simulink model "ElectricVehicleThermalManagementWithHeatPump_2026a_version"  (R2026a)
settings: Solver=VariableStepAuto  StopTime=3600  AbsTol=1e-3
PreLoadFcn:
  | init_nmpc
InitFcn:
  | init_nmpc
model workspace: external: MATLAB File ElectricVehicleThermalManagementWithHeatPumpParameters.m (data not in the file)
values from neighbouring files (symbols this model uses):
  battery_C1_LUT = [1913.6 12447 30609 ... (first row only)    [ElectricVehicleThermalManagementWithHeatPumpParameters.m]
  battery_capacity_LUT = [280.081 276.25 276.392]    [ElectricVehicleThermalManagementWithHeatPumpParameters.m]
  battery_cell_cp = 795    [ElectricVehicleThermalManagementWithHeatPumpParameters.m]
  battery_cell_mass = 2.5    [ElectricVehicleThermalManagementWithHeatPumpParameters.m]
  battery_Em_LUT = [3.4966 3.5057 3.5148 ... (first row only)    [ElectricVehicleThermalManagementWithHeatPumpParameters.m]
  battery_N_cells = 20    [ElectricVehicleThermalManagementWithHeatPumpParameters.m]
  battery_Qe_init = 0    [ElectricVehicleThermalManagementWithHeatPumpParameters.m]
  battery_R0_LUT = [0.0117 0.0085 0.009 ... (first row only)    [ElectricVehicleThermalManagementWithHeatPumpParameters.m]
  battery_R1_LUT = [0.0109 0.0029 0.0013 ... (first row only)    [ElectricVehicleThermalManagementWithHeatPumpParameters.m]
  battery_SOC_LUT = [0; 0.1; 0.25; 0.5; 0.75; 0.9; 1]    [ElectricVehicleThermalManagementWithHeatPumpParameters.m]
  battery_T_init = -5    [ElectricVehicleThermalManagementWithHeatPumpParameters.m]
  battery_temperature_LUT = [5 20 40]    [ElectricVehicleThermalManagementWithHeatPumpParameters.m]
  cabin_duct_area = 0.04    [ElectricVehicleThermalManagementWithHeatPumpParameters.m]
  cabin_T_init = -5    [ElectricVehicleThermalManagementWithHeatPumpParameters.m]
  chiller_area_primary = 0.43982297150257105    (= 0.439822971503)    [ElectricVehicleThermalManagementWithHeatPumpParameters.m]
  chiller_N_baffles = 3    [ElectricVehicleThermalManagementWithHeatPumpParameters.m]
  chiller_N_tubes = 100    [ElectricVehicleThermalManagementWithHeatPumpParameters.m]
  chiller_tube_D = 0.0035    [ElectricVehicleThermalManagementWithHeatPumpParameters.m]
  chiller_tube_L = 0.4    [ElectricVehicleThermalManagementWithHeatPumpParameters.m]
  chiller_wall_conductivity = 240    [ElectricVehicleThermalManagementWithHeatPumpParameters.m]
  chiller_wall_thickness = 0.0001    [ElectricVehicleThermalManagementWithHeatPumpParameters.m]
  cond_evap_air_area_flow = 0.3906    [ElectricVehicleThermalManagementWithHeatPumpParameters.m]
  cond_evap_air_area_primary = 1.4834999999999998    (= 1.4835)    [ElectricVehicleThermalManagementWithHeatPumpParameters.m]
  cond_evap_W = 0.015    [ElectricVehicleThermalManagementWithHeatPumpParameters.m]
  cond_evap_wall_conductivity = 240    [ElectricVehicleThermalManagementWithHeatPumpParameters.m]
  cond_evap_wall_thickness = 0.0001    [ElectricVehicleThermalManagementWithHeatPumpParameters.m]
  coolant_channel_D = 0.0092    [ElectricVehicleThermalManagementWithHeatPumpParameters.m]
  coolant_pipe_D = 0.019    [ElectricVehicleThermalManagementWithHeatPumpParameters.m]
  coolant_T_init = -5    [ElectricVehicleThermalManagementWithHeatPumpParameters.m]
  coolant_tank_area = 0.0121    [ElectricVehicleThermalManagementWithHeatPumpParameters.m]
  coolant_tank_volume = 1.25    [ElectricVehicleThermalManagementWithHeatPumpParameters.m]
  coolant_valve_D_ratio_max = 0.95    [ElectricVehicleThermalManagementWithHeatPumpParameters.m]
  coolant_valve_D_ratio_min = 0.001    [ElectricVehicleThermalManagementWithHeatPumpParameters.m]
  coolant_valve_displacement = 0.0063    [ElectricVehicleThermalManagementWithHeatPumpParameters.m]
  coolant_valve_S_max = 0.0053    [ElectricVehicleThermalManagementWithHeatPumpParameters.m]
  evaporator_air_area_flow = 0.12    [ElectricVehicleThermalManagementWithHeatPumpParameters.m]
  evaporator_air_area_primary = 0.4323    [ElectricVehicleThermalManagementWithHeatPumpParameters.m]
  evaporator_W = 0.015    [ElectricVehicleThermalManagementWithHeatPumpParameters.m]
  evaporator_wall_conductivity = 240    [ElectricVehicleThermalManagementWithHeatPumpParameters.m]
  evaporator_wall_thickness = 0.0001    [ElectricVehicleThermalManagementWithHeatPumpParameters.m]
  expansion_valve_D_ratio_max = 0.9    [ElectricVehicleThermalManagementWithHeatPumpParameters.m]
  hex_area_primary = 0.070371675440411369    (= 0.0703716754404)    [ElectricVehicleThermalManagementWithHeatPumpParameters.m]
  hex_N_tubes = 64    [ElectricVehicleThermalManagementWithHeatPumpParameters.m]
  hex_tube_D = 0.0035    [ElectricVehicleThermalManagementWithHeatPumpParameters.m]
  hex_wall_conductivity = 240    [ElectricVehicleThermalManagementWithHeatPumpParameters.m]
  hex_wall_thickness = 0.0001    [ElectricVehicleThermalManagementWithHeatPumpParameters.m]
  inner_cond_air_area_flow = 0.1953    [ElectricVehicleThermalManagementWithHeatPumpParameters.m]
  inner_cond_air_area_primary = 0.99520000000000008    (= 0.9952)    [ElectricVehicleThermalManagementWithHeatPumpParameters.m]
  inner_cond_W = 0.02    [ElectricVehicleThermalManagementWithHeatPumpParameters.m]
  inner_cond_wall_conductivity = 240    [ElectricVehicleThermalManagementWithHeatPumpParameters.m]
  inner_cond_wall_thickness = 0.0001    [ElectricVehicleThermalManagementWithHeatPumpParameters.m]
  pump_speed_max = 1000    [ElectricVehicleThermalManagementWithHeatPumpParameters.m]
  radiator_air_area_flow = 0.097499999999999989    (= 0.0975)    [ElectricVehicleThermalManagementWithHeatPumpParameters.m]
  radiator_air_area_primary = 0.43687499999999996    (= 0.436875)    [ElectricVehicleThermalManagementWithHeatPumpParameters.m]
  radiator_W = 0.015    [ElectricVehicleThermalManagementWithHeatPumpParameters.m]
  radiator_wall_conductivity = 240    [ElectricVehicleThermalManagementWithHeatPumpParameters.m]
  radiator_wall_thickness = 0.0001    [ElectricVehicleThermalManagementWithHeatPumpParameters.m]
  refrigerant_p_init = 0.25    [ElectricVehicleThermalManagementWithHeatPumpParameters.m]
  refrigerant_pipe_D = 0.01    [ElectricVehicleThermalManagementWithHeatPumpParameters.m]
  refrigerant_valve_D_ratio_max = 0.95    [ElectricVehicleThermalManagementWithHeatPumpParameters.m]
  refrigerant_valve_displacement = 0.005    [ElectricVehicleThermalManagementWithHeatPumpParameters.m]
libraries: fl_lib x227, nesl_utility x162, SimscapeFluids_lib x30, LiBatteryElements_lib x16, slpidlib x3, SignalEditorBlockLib x1
(part 12 of 13)

== system ElectricVehicleThermalManagementWithHeatPump_2026a_version/Battery/Pack 2/Thermal Model ==
  Battery Thermal Mass : fl_lib/Thermal/Thermal Elements/Thermal Mass  mass_type=foundation.enum.constant_variable.constant  mass=cell_mass*Ncells kg  sp_heat=cell_Cp_heat J/kg/K  mass_min=1e-6 kg  num_ports=foundation.enum.numPorts2.one  m_specify=off  m_priority=High  m=1 kg  m_nominal_specify=off  m_nominal_value=1  m_nominal_unit=kg  T_specify=on  T_priority=High  T=T_init K  T_nominal_specify=off  T_nominal_value=1  T_nominal_unit=K  Q_specify=off  Q_priority=None  Q=0 W  Q_nominal_specify=off  Q_nominal_value=1  Q_nominal_unit=W
  Controlled Heat Flow Rate Source : fl_lib/Thermal/Thermal Sources/Controlled Heat Flow Rate Source
  Temperature Sensor : fl_lib/Thermal/Thermal Sensors/Temperature Sensor  temperature_measure=foundation.enum.MeasurementReference.difference
  Thermal Reference : fl_lib/Thermal/Thermal Elements/Thermal Reference
  Thermal Reference2 : fl_lib/Thermal/Thermal Elements/Thermal Reference
  H : PMIOPort  Side=Left
  Pxn : PMIOPort  Port=2  Side=Left
  T : PMIOPort  Port=3  Side=Right
  connections:
  H/RConn1 -- Controlled Heat Flow Rate Source/LConn1 -- Battery Thermal Mass/LConn1 -- Temperature Sensor/LConn1
  Pxn/RConn1 -- Controlled Heat Flow Rate Source/RConn1
  Controlled Heat Flow Rate Source/RConn2 -- Thermal Reference2/LConn1
  Thermal Reference/LConn1 -- Temperature Sensor/RConn1
  T/RConn1 -- Temperature Sensor/RConn2

== system ElectricVehicleThermalManagementWithHeatPump_2026a_version/Battery/Pack 3/Lithium Cell 1RC ==
  note: Power
      | Losses
  C1 : LiBatteryElements_lib/C_table  C_Table=C1_LUT F  SOC_Table=SOC_LUT  Temp_Table=Temperature_LUT K  v0=0 V
  Em_table : LiBatteryElements_lib/Em_table  C_Table=Capacity_LUT hr*A  Em_Table=Em_LUT V  SOC_Table=SOC_LUT  Temp_Table=Temperature_LUT K  Qinit=Qe_init hr*A
  Power Sum : fl_lib/Physical Signals/Functions/PS Add
  R0 : LiBatteryElements_lib/R_table  R_Table=R0_LUT Ohm  SOC_Table=SOC_LUT  Temp_Table=Temperature_LUT K
  R1 : LiBatteryElements_lib/R_table  R_Table=R1_LUT Ohm  SOC_Table=SOC_LUT  Temp_Table=Temperature_LUT K
  P : PMIOPort  Side=Left
  + : PMIOPort  Port=2  Side=Left
  T : PMIOPort  Port=3  Side=Right
  - : PMIOPort  Port=4  Side=Right
  connections:
  R0/LConn3 -- R1/LConn3 -- Em_table/LConn3 -- C1/LConn3
  Em_table/RConn1 -- -/RConn1
  R0/LConn1 -- R1/RConn1 -- C1/RConn1
  R1/LConn1 -- C1/LConn1 -- Em_table/LConn1
  R1/LConn2 -- C1/LConn2 -- R0/LConn2 -- Em_table/RConn2 -- T/RConn1
  +/RConn1 -- R0/RConn1
  P/RConn1 -- Power Sum/RConn1
  Power Sum/LConn2 -- R0/RConn2
  R1/RConn2 -- Power Sum/LConn1

== system ElectricVehicleThermalManagementWithHeatPump_2026a_version/Battery/Pack 3/Thermal Model ==
  Battery Thermal Mass : fl_lib/Thermal/Thermal Elements/Thermal Mass  mass_type=foundation.enum.constant_variable.constant  mass=cell_mass*Ncells kg  sp_heat=cell_Cp_heat J/kg/K  mass_min=1e-6 kg  num_ports=foundation.enum.numPorts2.one  m_specify=off  m_priority=High  m=1 kg  m_nominal_specify=off  m_nominal_value=1  m_nominal_unit=kg  T_specify=on  T_priority=High  T=T_init K  T_nominal_specify=off  T_nominal_value=1  T_nominal_unit=K  Q_specify=off  Q_priority=None  Q=0 W  Q_nominal_specify=off  Q_nominal_value=1  Q_nominal_unit=W
  Controlled Heat Flow Rate Source : fl_lib/Thermal/Thermal Sources/Controlled Heat Flow Rate Source
  Temperature Sensor : fl_lib/Thermal/Thermal Sensors/Temperature Sensor  temperature_measure=foundation.enum.MeasurementReference.difference
  Thermal Reference : fl_lib/Thermal/Thermal Elements/Thermal Reference
  Thermal Reference2 : fl_lib/Thermal/Thermal Elements/Thermal Reference
  H : PMIOPort  Side=Left
  Pxn : PMIOPort  Port=2  Side=Left
  T : PMIOPort  Port=3  Side=Right
  connections:
  T/RConn1 -- Temperature Sensor/RConn2
  Thermal Reference/LConn1 -- Temperature Sensor/RConn1
  Controlled Heat Flow Rate Source/RConn2 -- Thermal Reference2/LConn1
  Pxn/RConn1 -- Controlled Heat Flow Rate Source/RConn1
  Temperature Sensor/LConn1 -- Battery Thermal Mass/LConn1 -- Controlled Heat Flow Rate Source/LConn1 -- H/RConn1

== system ElectricVehicleThermalManagementWithHeatPump_2026a_version/Battery/Pack 4/Lithium Cell 1RC ==
  note: Power
      | Losses
  C1 : LiBatteryElements_lib/C_table  C_Table=C1_LUT F  SOC_Table=SOC_LUT  Temp_Table=Temperature_LUT K  v0=0 V
  Em_table : LiBatteryElements_lib/Em_table  C_Table=Capacity_LUT hr*A  Em_Table=Em_LUT V  SOC_Table=SOC_LUT  Temp_Table=Temperature_LUT K  Qinit=Qe_init hr*A
  Power Sum : fl_lib/Physical Signals/Functions/PS Add
  R0 : LiBatteryElements_lib/R_table  R_Table=R0_LUT Ohm  SOC_Table=SOC_LUT  Temp_Table=Temperature_LUT K
  R1 : LiBatteryElements_lib/R_table  R_Table=R1_LUT Ohm  SOC_Table=SOC_LUT  Temp_Table=Temperature_LUT K
  P : PMIOPort  Side=Left
  + : PMIOPort  Port=2  Side=Left
  T : PMIOPort  Port=3  Side=Right
  - : PMIOPort  Port=4  Side=Right
  connections:
  R1/RConn2 -- Power Sum/LConn1
  Power Sum/LConn2 -- R0/RConn2
  P/RConn1 -- Power Sum/RConn1
  +/RConn1 -- R0/RConn1
  T/RConn1 -- Em_table/RConn2 -- R0/LConn2 -- C1/LConn2 -- R1/LConn2
  Em_table/LConn1 -- C1/LConn1 -- R1/LConn1
  C1/RConn1 -- R1/RConn1 -- R0/LConn1
  Em_table/RConn1 -- -/RConn1
  C1/LConn3 -- Em_table/LConn3 -- R1/LConn3 -- R0/LConn3

== system ElectricVehicleThermalManagementWithHeatPump_2026a_version/Battery/Pack 4/Thermal Model ==
  Battery Thermal Mass : fl_lib/Thermal/Thermal Elements/Thermal Mass  mass_type=foundation.enum.constant_variable.constant  mass=cell_mass*Ncells kg  sp_heat=cell_Cp_heat J/kg/K  mass_min=1e-6 kg  num_ports=foundation.enum.numPorts2.one  m_specify=off  m_priority=High  m=1 kg  m_nominal_specify=off  m_nominal_value=1  m_nominal_unit=kg  T_specify=on  T_priority=High  T=T_init K  T_nominal_specify=off  T_nominal_value=1  T_nominal_unit=K  Q_specify=off  Q_priority=None  Q=0 W  Q_nominal_specify=off  Q_nominal_value=1  Q_nominal_unit=W
  Controlled Heat Flow Rate Source : fl_lib/Thermal/Thermal Sources/Controlled Heat Flow Rate Source
  Temperature Sensor : fl_lib/Thermal/Thermal Sensors/Temperature Sensor  temperature_measure=foundation.enum.MeasurementReference.difference
  Thermal Reference : fl_lib/Thermal/Thermal Elements/Thermal Reference
  Thermal Reference2 : fl_lib/Thermal/Thermal Elements/Thermal Reference
  H : PMIOPort  Side=Left
  Pxn : PMIOPort  Port=2  Side=Left
  T : PMIOPort  Port=3  Side=Right
  connections:
  H/RConn1 -- Controlled Heat Flow Rate Source/LConn1 -- Battery Thermal Mass/LConn1 -- Temperature Sensor/LConn1
  Pxn/RConn1 -- Controlled Heat Flow Rate Source/RConn1
  Controlled Heat Flow Rate Source/RConn2 -- Thermal Reference2/LConn1
  Thermal Reference/LConn1 -- Temperature Sensor/RConn1
  T/RConn1 -- Temperature Sensor/RConn2

== system ElectricVehicleThermalManagementWithHeatPump_2026a_version/Controls/Cabin Air Control/Blower Control ==
  T_cabin : Inport
  T_cabin_sp : Inport  Port=2
  T_env : Inport  Port=3
  PID Controller : slpidlib/PID Controller  Controller=PI  Form=Parallel  TimeDomain=Continuous-time  UseExternalTs=off  SampleTime=-1  IntegratorMethod=Forward Euler  FilterMethod=Forward Euler  ControllerParametersSource=internal  P=0.5  I=2e-3  UseKiTs=off  D=0  UseExternalDerivativeSource=off  N=100  UseFilter=on  TunerSelectOption=Transfer Function Based (PID Tuner App)  ZeroCross=off  InitialConditionSource=internal  InitialConditionForIntegrator=0  InitialConditionForFilter=0  DifferentiatorICPrevScaledInput=0  ExternalReset=either  TrackingMode=off  Kt=1  LimitOutput=on  SatLimitsSource=internal  UpperSaturationLimit=1  LowerSaturationLimit=0  LinearizeAsGain=on  AntiWindupMode=back-calculation  Kb=1  LimitIntegrator=off  UpperIntegratorSaturationLimit=inf  LowerIntegratorSaturationLimit=-inf  POutMin=[]  POutMax=[]  IOutMin=[]  IOutMax=[]  DOutMin=[]  DOutMax=[]  NOutMin=[]  NOutMax=[]  SumOutMin=[]  SumOutMax=[]  SaturationOutMin=[]  SaturationOutMax=[]  PParamMin=[]  PParamMax=[]  IParamMin=[]  IParamMax=[]  DParamMin=[]  DParamMax=[]  NParamMin=[]  NParamMax=[]  KbParamMin=[]  KbParamMax=[]  KtParamMin=[]  KtParamMax=[]  KbOutMin=[]  KbOutMax=[]  KtOutMin=[]  KtOutMax=[]  IntegratorOutMin=[]  IntegratorOutMax=[]  FilterOutMin=[]  FilterOutMax=[]  SumI1OutMin=[]  SumI1OutMax=[]  SumI2OutMin=[]  SumI2OutMax=[]  SumI3OutMin=[]  SumI3OutMax=[]  SumI4OutMin=[]  SumI4OutMax=[]  SumDOutMin=[]  SumDOutMax=[]  DifferentiatorOutMin=[]  DifferentiatorOutMax=[]  FilterDiffOutCoefMin=[]  FilterDiffOutCoefMax=[]  ReciprocalOutMin=[]  ReciprocalOutMax=[]  SumDenOutMin=[]  SumDenOutMax=[]  SumNumOutMin=[]  SumNumOutMax=[]  DivideOutMin=[]  DivideOutMax=[]  UdiffTsProdOutMin=[]  UdiffTsProdOutMax=[]  NTsProdOutMin=[]  NTsProdOutMax=[]  UintegralTsProdOutMin=[]  UintegralTsProdOutMax=[]  UngainTsProdOutMin=[]  UngainTsProdOutMax=[]  ClampingZeroOutDataTypeStr=Inherit: Inherit via back propagation  ClampingZeroOutMin=[]  ClampingZeroOutMax=[]  FilterDenConstantOutDataTypeStr=Inherit: Inherit via back propagation  FilterDenConstantOutMin=[]  FilterDenConstantOutMax=[]  PCopyOutDataTypeStr=Inherit: Inherit via back propagation  PCopyOutMin=[]  PCopyOutMax=[]  NCopyOutDataTypeStr=Inherit: Inherit via back propagation  NCopyOutMin=[]  NCopyOutMax=[]  IntegratorContinuousStateAttributes=''  IntegratorStateMustResolveToSignalObject=off  IntegratorRTWStateStorageClass=Auto  FilterContinuousStateAttributes=''  FilterStateMustResolveToSignalObject=off  FilterRTWStateStorageClass=Auto  ParallelPVariant=InternalParameters  IdealPVariant=Disabled  IVariant=InternalParameters  DVariant=Disabled  IntegratorVariant=Continuous  SatVariant=Enabled  AWVariant=BackCalculation  PCopyVariant=Disabled  TRVariant=Disabled  FdbkBlocksVariant=Forward  IdealPFdbkVariant=Disabled  SatFdbkVariant=Disabled  DerivativeFilterVariant=Disabled  NVariant=Disabled  NCopyVariant=Disabled_SignalSpec  FilterICVariant=Disabled  IntegratorICVariant=InternalICs  ExternalResetVariant=ExternalReset  TRSumVariant=Passthrough  SumFdbkVariant=Disabled  SumVariant=Sum_PI  TsampFilterVariant=InternalTs  TsampNgainVariant=Passthrough  TsampIntegralVariant=Disabled_SignalSpec  ExternalSaturationOutDataTypeStr=Inherit: Same as second input  DerivativeSourceVariant=Disabled  PreIntVariant=InternalPreInt
  Product : Product
  Sign : Signum
  Sum : Sum  Inputs=-+|
  Sum1 : Sum  Inputs=-+|
  cmd_blower : Outport
  wires:
  T_cabin/1 -> Sum/2
  Sum/1 -> Product/1
  PID Controller/1 -> cmd_blower/1
  T_env/1 -> Sum1/2
  Sign/1 -> PID Controller/2, Product/2
  Product/1 -> PID Controller/1
  Sum1/1 -> Sign/1
  T_cabin_sp/1 -> Sum1/1, Sum/1

== system ElectricVehicleThermalManagementWithHeatPump_2026a_version/Controls/Cabin Air Control/Comfort ==
  T_cabin : Inport
  T_desired : Inport  Port=2
  T_env : Inport  Port=3
  Bias : Bias  Bias=-21  SaturateOnIntegerOverflow=off
  Correction : Lookup_n-D  NumberOfTableDimensions=1  BreakpointsForDimension1=[-100 -10 0 10 100]  BeginIndexSearchUsingPreviousIndexResult=on  Table=[20 15 0 -15 -20]  InternalRulePriority=Speed  RndMeth=Simplest
  Gain : Gain
  Recirculation : Lookup_n-D  NumberOfTableDimensions=1  BreakpointsForDimension1=|  BeginIndexSearchUsingPreviousIndexResult=on  Table=[1 0.9 0.5 0 0.2 0.9 1]  ExtrapMethod=Clip  InternalRulePriority=Speed  RndMeth=Simplest
      | [-20
      | -10
      | 0
      | 20
      | 30
      | 40
      | 50]
  Scope : Scope
      settings: ActiveDisplayYMinimum=11.5  ActiveDisplayYMaximum=31.5
  Sum : Sum  Inputs=|+-
  Sum1 : Sum  Inputs=++|
  Sum2 : Sum  Inputs=++|
  Target Cabin Temperature : Lookup_n-D  NumberOfTableDimensions=1  BreakpointsForDimension1=|  BeginIndexSearchUsingPreviousIndexResult=on  Table=[25 24 23 22 21 20 19 19]  InternalRulePriority=Speed  RndMeth=Simplest
      | [-40
      | -20
      | 0
      | 20
      | 30
      | 40
      | 50
      | 80]
  Target Vent Temperature : Lookup_n-D  NumberOfTableDimensions=1  BreakpointsForDimension1=|  BeginIndexSearchUsingPreviousIndexResult=on  Table=[65 52 36 21 14 7 3 3]  InternalRulePriority=Speed  RndMeth=Simplest
      | [-40
      | -20
      | 0
      | 20
      | 30
      | 40
      | 50
      | 80]
  T_cabin_sp : Outport
  T_vent_sp : Outport  Port=2
  cmd_recirc : Outport  Port=3
  wires:
  T_env/1 -> Recirculation/1, Target Vent Temperature/1, Target Cabin Temperature/1
  T_cabin/1 -> Sum/1
  Sum/1 -> Gain/1
  Gain/1 -> Correction/1
  Sum1/1 -> T_vent_sp/1
  Correction/1 -> Sum1/1
  Target Vent Temperature/1 -> Sum1/2
  Recirculation/1 -> cmd_recirc/1
  Sum2/1 -> Sum/2
  Target Cabin Temperature/1 -> Sum2/2
  T_desired/1 -> T_cabin_sp/1, Bias/1
  Bias/1 -> Sum2/1

== system ElectricVehicleThermalManagementWithHeatPump_2026a_version/Controls/Coolant Loop Control/Battery Pump Control ==
  cmd_motor_pump : Inport
  T_battery : Inport  Port=2
  cmd_parallel_serial : Inport  Port=3
  Relay : Relay  OnSwitchValue=45  OffSwitchValue=40  OffOutputValue=0.5
  Switch : Switch  Criteria=u2 > Threshold  Threshold=0.5  SaturateOnIntegerOverflow=off  InputSameDT=off
  cmd_battery_pump : Outport
  wires:
  T_battery/1 -> Relay/1
  cmd_parallel_serial/1 -> Switch/2
  Switch/1 -> cmd_battery_pump/1
  Relay/1 -> Switch/3
  cmd_motor_pump/1 -> Switch/1

== system ElectricVehicleThermalManagementWithHeatPump_2026a_version/Controls/Coolant Loop Control/Motor Pump Control ==
  T_motor : Inport
  1-D Lookup Table : Lookup_n-D  NumberOfTableDimensions=1  BreakpointsForDimension1=[-50 45 48 52 58 60 75 130]  IndexSearchMethod=Linear search  BeginIndexSearchUsingPreviousIndexResult=on  Table=[0 0 0.1 0.3 0.5 0.7 1 1]  ExtrapMethod=Clip  InternalRulePriority=Speed  RndMeth=Simplest
  Saturation : Saturate  UpperLimit=1  LowerLimit=0.3  ZeroCross=off
  cmd_motor_pump : Outport
  wires:
  T_motor/1 -> 1-D Lookup Table/1
  1-D Lookup Table/1 -> Saturation/1
  Saturation/1 -> cmd_motor_pump/1

== system ElectricVehicleThermalManagementWithHeatPump_2026a_version/Controls/Coolant Loop Control/Parallel-Serial Mode ==
  note: 0 = Parallel mode
      |
      | 1 = Serial mode
  thermal_mode : Inport
  T_env : Inport  Port=2
  T_coolant_inverter_out : Inport  Port=3
  Constant : Constant
  MinMax : MinMax  Function=max  Inputs=2  ZeroCross=off
  Relay : Relay  OnSwitchValue=35  OffSwitchValue=30  OnOutputValue=0  OffOutputValue=1
  Switch : Switch  Criteria=u2 > Threshold  Threshold=1  SaturateOnIntegerOverflow=off  InputSameDT=off
  cmd_parallel_serial : Outport
  wires:
  T_env/1 -> MinMax/1
  T_coolant_inverter_out/1 -> MinMax/2
  MinMax/1 -> Relay/1
  Switch/1 -> cmd_parallel_serial/1
  thermal_mode/1 -> Switch/2
  Constant/1 -> Switch/1
  Relay/1 -> Switch/3

== system ElectricVehicleThermalManagementWithHeatPump_2026a_version/Controls/Fan Control/Condenser Requirement ==
  p_cond : Inport
  T_env : Inport  Port=2
  1-D Lookup Table : Lookup_n-D  NumberOfTableDimensions=1  BreakpointsForDimension1=[0 20 30 40 50]  IndexSearchMethod=Linear search  BeginIndexSearchUsingPreviousIndexResult=on  Table=[2.0 2.0 1.8 1.5 1.3]  InternalRulePriority=Speed  RndMeth=Simplest
  1-D Lookup Table1 : Lookup_n-D  NumberOfTableDimensions=1  BreakpointsForDimension1=[0 20 30 40 50]  IndexSearchMethod=Linear search  BeginIndexSearchUsingPreviousIndexResult=on  Table=[1.4 1.4 1.3 1.2 1.1]  InternalRulePriority=Speed  RndMeth=Simplest
  1-D Lookup Table2 : Lookup_n-D  NumberOfTableDimensions=1  BreakpointsForDimension1=[0 20 30 40 50]  IndexSearchMethod=Linear search  BeginIndexSearchUsingPreviousIndexResult=on  Table=[0.8 0.8 0.8 0.8 0.8]  InternalRulePriority=Speed  RndMeth=Simplest
  Bias : Bias  Bias=0.4  SaturateOnIntegerOverflow=off
  Bias1 : Bias  Bias=0.4  SaturateOnIntegerOverflow=off
  Bias2 : Bias  Bias=0.3  SaturateOnIntegerOverflow=off
  Relay Level 1 : Subsystem
  Relay Level 2 : Subsystem
  Relay Level 3 : Subsystem
  Scope : Scope
      settings: DataLoggingVariableName=ScopeData4
  Scope1 : Scope
      settings: DataLoggingVariableName=ScopeData5
  Sum : Sum  Inputs=+++
  req : Outport
  wires:
  Sum/1 -> Scope/1, req/1
  p_cond/1 -> Scope1/1, Relay Level 3/1(in), Relay Level 2/1(in), Relay Level 1/1(in)
  Relay Level 3/1(out) -> Sum/1
  Relay Level 2/1(out) -> Sum/2
  Relay Level 1/1(out) -> Sum/3
  1-D Lookup Table/1 -> Relay Level 3/3(low), Bias/1
  Bias/1 -> Relay Level 3/2(high)
  1-D Lookup Table1/1 -> Relay Level 2/3(low), Bias1/1
  Bias1/1 -> Relay Level 2/2(high)
  1-D Lookup Table2/1 -> Relay Level 1/3(low), Bias2/1
  Bias2/1 -> Relay Level 1/2(high)
  T_env/1 -> 1-D Lookup Table/1, 1-D Lookup Table1/1, 1-D Lookup Table2/1

== system ElectricVehicleThermalManagementWithHeatPump_2026a_version/Controls/Fan Control/Inverter Requirement ==
  T_inverter : Inport
  Gain : Gain  Gain=1/3
  Relay Level 1 : Relay  OnSwitchValue=75  OffSwitchValue=65
  Relay Level 2 : Relay  OnSwitchValue=85  OffSwitchValue=76
  Relay Level 3 : Relay  OnSwitchValue=95  OffSwitchValue=86
  Sum : Sum  Inputs=+++
  cmd_fan : Outport
  wires:
  T_inverter/1 -> Relay Level 1/1, Relay Level 3/1, Relay Level 2/1
  Relay Level 2/1 -> Sum/2
  Relay Level 3/1 -> Sum/1
  Relay Level 1/1 -> Sum/3
  Sum/1 -> Gain/1
  Gain/1 -> cmd_fan/1

== system ElectricVehicleThermalManagementWithHeatPump_2026a_version/Controls/Fan Control/Motor Requirement ==
  T_motor : Inport
  1-D Lookup Table : Lookup_n-D  NumberOfTableDimensions=1  BreakpointsForDimension1=[-50 35 38 42 48 50 65 130]  IndexSearchMethod=Linear search  BeginIndexSearchUsingPreviousIndexResult=on  Table=[0 0 0.1 0.3 0.5 0.7 1 1]  InternalRulePriority=Speed  RndMeth=Simplest
  cmd_fan : Outport
  wires:
  T_motor/1 -> 1-D Lookup Table/1
  1-D Lookup Table/1 -> cmd_fan/1

== system ElectricVehicleThermalManagementWithHeatPump_2026a_version/Controls/Fan Control/Vehicle Speed Requirement ==
  v_vehicle : Inport
  Add : Sum  Inputs=++++
  Relay Level 1 : Relay  OnSwitchValue=20  OffSwitchValue=15
  Relay Level 2 : Relay  OnSwitchValue=60  OffSwitchValue=55
  Relay Level 3 : Relay  OnSwitchValue=75  OffSwitchValue=65
  Relay Level 4 : Relay  OnSwitchValue=90  OffSwitchValue=80
  req : Outport
  wires:
  Relay Level 4/1 -> Add/1
  Relay Level 3/1 -> Add/2
  Relay Level 2/1 -> Add/3
  Relay Level 1/1 -> Add/4
  Add/1 -> req/1
  v_vehicle/1 -> Relay Level 2/1, Relay Level 1/1, Relay Level 3/1, Relay Level 4/1

== system ElectricVehicleThermalManagementWithHeatPump_2026a_version/Controls/Thermal Mode/Mode Selection ==
  note: 0 = Off
      |
      | 1 = Cold loop
      |
      | 2 = Heat pump
  T_env : Inport
  Constant : Constant
  Constant1 : Constant  Value=0
  Constant2 : Constant  Value=2
  Switch : Switch  Criteria=u2 > Threshold  Threshold=19  SaturateOnIntegerOverflow=off  InputSameDT=off
  Switch1 : Switch  Threshold=21  SaturateOnIntegerOverflow=off  InputSameDT=off
  setpoint : Outport
  wires:
  T_env/1 -> Switch/2, Switch1/2
  Switch/1 -> setpoint/1
  Switch1/1 -> Switch/1
  Constant/1 -> Switch1/1
  Constant1/1 -> Switch1/3
  Constant2/1 -> Switch/3

== system ElectricVehicleThermalManagementWithHeatPump_2026a_version/Controls/Thermal Mode/Mode Transition ==
  note: 0 = Off
      |
      | 1 = Cold loop
      |
      | 2 = Heat pump
  setpoint : Inport
  rpm_comp : Inport  Port=2
  Memory : Memory
  Switch : Switch  Criteria=u2 > Threshold  SaturateOnIntegerOverflow=off  InputSameDT=off
  Transition from off to operating : Subsystem
  Transition from operating to off : Subsystem
  thermal_mode : Outport
  wires:
  setpoint/1 -> Transition from operating to off/2(setpoint), Transition from off to operating/1(setpoint)
  Transition from operating to off/1(mode) -> Switch/1
  Transition from off to operating/1(mode) -> Switch/3
  Memory/1 -> Transition from operating to off/1(current), Switch/2
  Switch/1 -> Memory/1, thermal_mode/1
  rpm_comp/1 -> Transition from off to operating/2(rpm_comp)

== system ElectricVehicleThermalManagementWithHeatPump_2026a_version/Controls/Valves Control/Chiller Expansion Valve ==
  thermal_mode : Inport
  T_coolant_battery_in : Inport  Port=2
  Constant : Constant  Value=0
  Constant1 : Constant  Value=0
  Multiport Switch : MultiPortSwitch  DataPortOrder=Zero-based contiguous  zeroidx=on  SaturateOnIntegerOverflow=off  InputSameDT=off
  Relay : Relay  OnSwitchValue=35  OffSwitchValue=25  OnOutputValue=0.024
  Scope : Scope
      settings: ActiveDisplayYMinimum=0.014  ActiveDisplayYMaximum=0.034
  Scope1 : Scope
      settings: ActiveDisplayYMinimum=-0.003  ActiveDisplayYMaximum=0.027  DataLoggingVariableName=ScopeData2
  Transfer Fcn : TransferFcn  Denominator=[30 1]
  cmd_exv_chiller : Outport
  wires:
  thermal_mode/1 -> Multiport Switch/1
  Multiport Switch/1 -> cmd_exv_chiller/1
  Constant/1 -> Multiport Switch/2
  Constant1/1 -> Multiport Switch/4
  Transfer Fcn/1 -> Scope1/1, Multiport Switch/3
  Relay/1 -> Scope/1, Transfer Fcn/1
  T_coolant_battery_in/1 -> Relay/1

== system ElectricVehicleThermalManagementWithHeatPump_2026a_version/Controls/Valves Control/Evaporator Expansion Valve ==
  thermal_mode : Inport
  T_env : Inport  Port=2
  1-D Lookup Table : Lookup_n-D  NumberOfTableDimensions=1  BreakpointsForDimension1=[20 40]  BeginIndexSearchUsingPreviousIndexResult=on  Table=[0.006 0.009]  ExtrapMethod=Clip  InternalRulePriority=Speed  RndMeth=Simplest
  Constant : Constant  Value=0
  Constant1 : Constant  Value=0
  Multiport Switch : MultiPortSwitch  DataPortOrder=Zero-based contiguous  zeroidx=on  SaturateOnIntegerOverflow=off  InputSameDT=off
  cmd_exv_evap : Outport
  wires:
  thermal_mode/1 -> Multiport Switch/1
  Multiport Switch/1 -> cmd_exv_evap/1
  Constant/1 -> Multiport Switch/2
  Constant1/1 -> Multiport Switch/4
  1-D Lookup Table/1 -> Multiport Switch/3
  T_env/1 -> 1-D Lookup Table/1

== system ElectricVehicleThermalManagementWithHeatPump_2026a_version/Controls/Valves Control/Heat Pump Expansion Valve ==
  thermal_mode : Inport
  T_env : Inport  Port=2
  1-D Lookup Table : Lookup_n-D  NumberOfTableDimensions=1  BreakpointsForDimension1=[-10 0]  BeginIndexSearchUsingPreviousIndexResult=on  Table=[0.007 0.006]  ExtrapMethod=Clip  InternalRulePriority=Speed  RndMeth=Simplest
  Constant : Constant  Value=0
  Constant1 : Constant
  Multiport Switch : MultiPortSwitch  DataPortOrder=Zero-based contiguous  zeroidx=on  SaturateOnIntegerOverflow=off  InputSameDT=off
  Scope : Scope
      settings: ActiveDisplayYMinimum=0.006  ActiveDisplayYMaximum=0.008
  Scope1 : Scope
      settings: DataLoggingVariableName=ScopeData2
  cmd_exv_heatpump : Outport
  wires:
  thermal_mode/1 -> Scope1/1, Multiport Switch/1
  Multiport Switch/1 -> Scope/1, cmd_exv_heatpump/1
  Constant/1 -> Multiport Switch/2
  Constant1/1 -> Multiport Switch/3
  1-D Lookup Table/1 -> Multiport Switch/4
  T_env/1 -> 1-D Lookup Table/1

== system ElectricVehicleThermalManagementWithHeatPump_2026a_version/Controls/Valves Control/Radiator 3-Way Valve ==
  thermal_mode : Inport
  T_coolant_inverter_out : Inport  Port=2
  Constant : Constant  Value=0
  Memory : Memory
  Multiport Switch : MultiPortSwitch  DataPortOrder=Zero-based contiguous  zeroidx=on  SaturateOnIntegerOverflow=off  InputSameDT=off
  Relay : Relay  OnSwitchValue=50  OffSwitchValue=25  OnOutputValue=0  OffOutputValue=1
  Scope : Scope
      settings: ActiveDisplayYMinimum=-10.31389  ActiveDisplayYMaximum=-7.17501
  Scope1 : Scope
      settings: ActiveDisplayYMinimum=0.9  ActiveDisplayYMaximum=1.1
  cmd_rad_bypass : Outport
  wires:
  thermal_mode/1 -> Multiport Switch/1
  Relay/1 -> Scope1/1, Multiport Switch/4
  Constant/1 -> Multiport Switch/3
  Memory/1 -> Multiport Switch/2
  T_coolant_inverter_out/1 -> Scope/1, Relay/1
  Multiport Switch/1 -> Memory/1, cmd_rad_bypass/1

== system ElectricVehicleThermalManagementWithHeatPump_2026a_version/Controls/Valves Control/Refrigerant and Air 3-Way Valve ==
  thermal_mode : Inport
  Constant : Constant  Value=0
  Constant1 : Constant
  Memory : Memory
  Multiport Switch : MultiPortSwitch  DataPortOrder=Zero-based contiguous  zeroidx=on  SaturateOnIntegerOverflow=off  InputSameDT=off
  Scope : Scope
      settings: DataLoggingVariableName=ScopeData15
  Scope1 : Scope
      settings: ActiveDisplayYMinimum=0.9  ActiveDisplayYMaximum=1.1  DataLoggingVariableName=ScopeData16
  cmd_refrig_bypass : Outport
  cmd_blend_air : Outport  Port=2
  wires:
  thermal_mode/1 -> Scope/1, Multiport Switch/1
  Constant1/1 -> Multiport Switch/4
  Constant/1 -> Multiport Switch/3
  Multiport Switch/1 -> Scope1/1, cmd_blend_air/1, Memory/1, cmd_refrig_bypass/1
  Memory/1 -> Multiport Switch/2

== system ElectricVehicleThermalManagementWithHeatPump_2026a_version/Scenario/Power Demand/Derivative ==
  V : Inport
  Gain : Gain  Gain=1/tau
  Integrator : Integrator
  Sum : Sum  Inputs=|+-
  A : Outport
  wires:
  V/1 -> Sum/1
  Sum/1 -> Gain/1
  Gain/1 -> Integrator/1, A/1
  Integrator/1 -> Sum/2

== system ElectricVehicleThermalManagementWithHeatPump_2026a_version/Controls/Fan Control/Condenser Requirement/Relay Level 1 ==
  in : Inport
  high : Inport  Port=2
  low : Inport  Port=3
  Data Type Conversion : DataTypeConversion  SaturateOnIntegerOverflow=off  RndMeth=Floor
  Relational Operator : RelationalOperator  OutDataTypeStr=boolean  RndMeth=Simplest  InputSameDT=off
  Relational Operator1 : RelationalOperator  Operator=>  OutDataTypeStr=boolean  RndMeth=Simplest  InputSameDT=off
  Relay : Relay  OnSwitchValue=1.5  OffSwitchValue=0.5
  Sum : Sum  Inputs=|++
  out : Outport
  wires:
  Sum/1 -> Data Type Conversion/1
  Data Type Conversion/1 -> Relay/1
  Relational Operator1/1 -> Sum/2
  Relational Operator/1 -> Sum/1
  Relay/1 -> out/1
  low/1 -> Relational Operator1/2
  high/1 -> Relational Operator/2
  in/1 -> Relational Operator/1, Relational Operator1/1

== system ElectricVehicleThermalManagementWithHeatPump_2026a_version/Controls/Fan Control/Condenser Requirement/Relay Level 2 ==
  in : Inport
  high : Inport  Port=2
  low : Inport  Port=3
  Data Type Conversion : DataTypeConversion  SaturateOnIntegerOverflow=off  RndMeth=Floor
  Relational Operator : RelationalOperator  OutDataTypeStr=boolean  RndMeth=Simplest  InputSameDT=off
  Relational Operator1 : RelationalOperator  Operator=>  OutDataTypeStr=boolean  RndMeth=Simplest  InputSameDT=off
  Relay : Relay  OnSwitchValue=1.5  OffSwitchValue=0.5
  Sum : Sum  Inputs=|++
  out : Outport
  wires:
  Sum/1 -> Data Type Conversion/1
  Data Type Conversion/1 -> Relay/1
  Relational Operator1/1 -> Sum/2
  Relational Operator/1 -> Sum/1
  Relay/1 -> out/1
  low/1 -> Relational Operator1/2
  high/1 -> Relational Operator/2
  in/1 -> Relational Operator/1, Relational Operator1/1

== system ElectricVehicleThermalManagementWithHeatPump_2026a_version/Controls/Fan Control/Condenser Requirement/Relay Level 3 ==
  in : Inport
  high : Inport  Port=2
  low : Inport  Port=3
  Data Type Conversion : DataTypeConversion  SaturateOnIntegerOverflow=off  RndMeth=Floor
  Relational Operator : RelationalOperator  OutDataTypeStr=boolean  RndMeth=Simplest  InputSameDT=off
  Relational Operator1 : RelationalOperator  Operator=>  OutDataTypeStr=boolean  RndMeth=Simplest  InputSameDT=off
  Relay : Relay  OnSwitchValue=1.5  OffSwitchValue=0.5
  Sum : Sum  Inputs=|++
  out : Outport
  wires:
  Sum/1 -> Data Type Conversion/1
  Data Type Conversion/1 -> Relay/1
  Relational Operator1/1 -> Sum/2
  Relational Operator/1 -> Sum/1
  Relay/1 -> out/1
  low/1 -> Relational Operator1/2
  high/1 -> Relational Operator/2
  in/1 -> Relational Operator/1, Relational Operator1/1

== system ElectricVehicleThermalManagementWithHeatPump_2026a_version/Controls/Thermal Mode/Mode Transition/Transition from off to operating ==
  setpoint : Inport
  rpm_comp : Inport  Port=2
  Constant : Constant  Value=0
  Switch : Switch  Criteria=u2 > Threshold  Threshold=10  SaturateOnIntegerOverflow=off  InputSameDT=off
  mode : Outport
  wires:
  rpm_comp/1 -> Switch/2
  Switch/1 -> mode/1
  Constant/1 -> Switch/1
  setpoint/1 -> Switch/3

== system ElectricVehicleThermalManagementWithHeatPump_2026a_version/Controls/Thermal Mode/Mode Transition/Transition from operating to off ==
  current : Inport
  setpoint : Inport  Port=2
  Constant : Constant  Value=0
  Relational Operator : RelationalOperator  Operator=~=  OutDataTypeStr=boolean  RndMeth=Simplest  InputSameDT=off
  Switch : Switch  Criteria=u2 ~= 0  SaturateOnIntegerOverflow=off  InputSameDT=off
  mode : Outport
  wires:
  Relational Operator/1 -> Switch/2
  current/1 -> Relational Operator/1
  setpoint/1 -> Switch/3, Relational Operator/2
  Switch/1 -> mode/1
  Constant/1 -> Switch/1
